simulink model "Cerano23210696Pr4"  (R2023a)
settings: Solver=ode15s  StartTime=0.0  StopTime=10.0  MaxStep=1E-3  RelTol=1e-3
libraries: fl_lib x14, nesl_utility x6, slpidlib x1
settings Model: LastModifiedBy=David
settings DataIOCC: SaveFormat=Array  ReturnWorkspaceOutputs=off  TimeSaveName=t
settings DebuggingCC: AlgebraicLoopMsg=none  ArtificialAlgebraicLoopMsg=none  MaxConsecutiveZCsMsg=none  ModelReferenceExtraNoncontSigs=none  OperatingPointInterfaceChecksumMismatchMsg=none
settings RTWCC: GPUComputeCapability=5.0

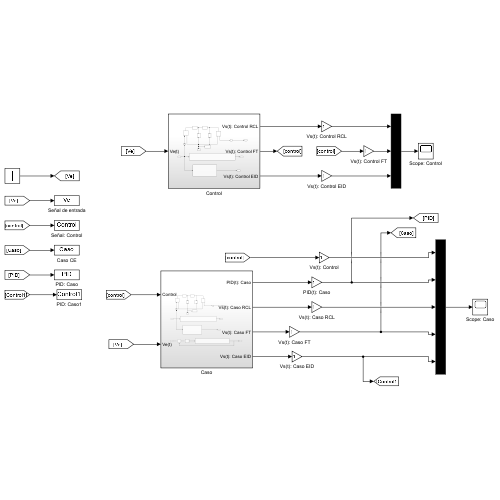
[thumbnail: Simulink's stored preview of the top-level diagram]
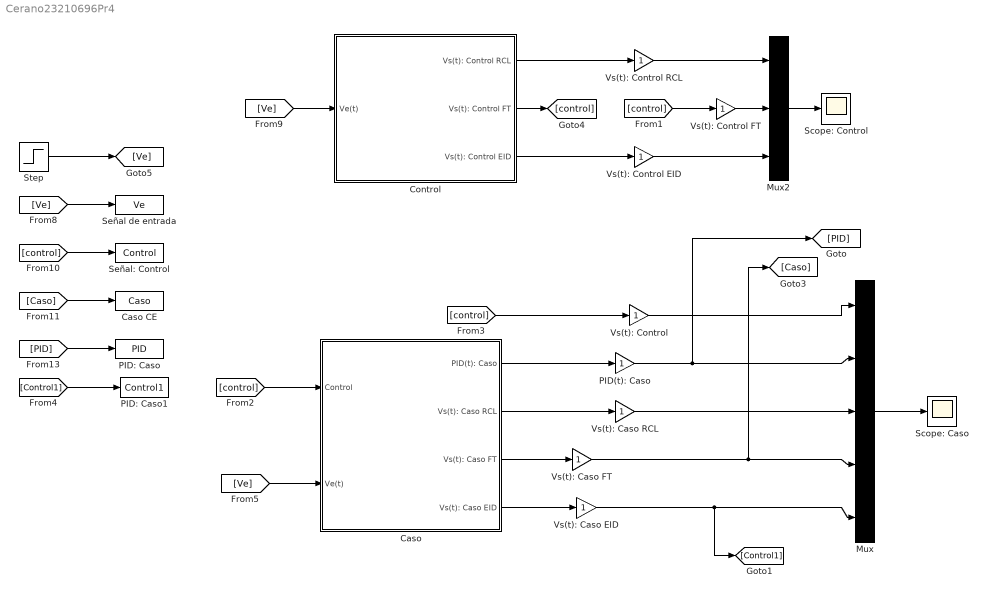
== system Cerano23210696Pr4 ==
  Caso : Subsystem
  Caso CE : ToWorkspace  VariableName=Caso  SampleTime=-1
  Control : Subsystem
  Mux : Mux  Inputs=5
  Mux2 : Mux  Inputs=3
  PID(t): Caso : Gain
  PID: Caso : ToWorkspace  VariableName=PID  SampleTime=-1
  PID: Caso1 : ToWorkspace  VariableName=Control1  SampleTime=-1
  Scope: Caso : Scope
  Scope: Control : Scope
  Señal de entrada : ToWorkspace  VariableName=Ve  SampleTime=-1
  Señal: Control : ToWorkspace  VariableName=Control  SampleTime=-1
  Step : Step  Time=0  SampleTime=0
  Vs(t): Caso EID : Gain
  Vs(t): Caso FT : Gain
  Vs(t): Caso RCL : Gain
  Vs(t): Control : Gain
  Vs(t): Control EID : Gain
  Vs(t): Control FT : Gain
  Vs(t): Control RCL : Gain
  wires:
  Mux/1 -> Scope: Caso/1
  [control] -> Caso/1(Control)
  [Ve] -> Caso/2(Ve(t))
  Mux2/1 -> Scope: Control/1
  [control] -> Vs(t): Control FT/1
  [Ve] -> Señal de entrada/1
  [control] -> Señal: Control/1
  [Caso] -> Caso CE/1
  [PID] -> PID: Caso/1
  Step/1 -> [Ve]
  Vs(t): Control FT/1 -> Mux2/2
  Vs(t): Control RCL/1 -> Mux2/1
  Control/1(Vs(t): Control RCL) -> Vs(t): Control RCL/1
  Control/2(Vs(t): Control FT) -> [control]
  [Ve] -> Control/1(Ve(t))
  Control/3(Vs(t): Control EID) -> Vs(t): Control EID/1
  Vs(t): Control EID/1 -> Mux2/3
  [control] -> Vs(t): Control/1
  Vs(t): Control/1 -> Mux/1
  Caso/2(Vs(t): Caso RCL) -> Vs(t): Caso RCL/1
  Vs(t): Caso RCL/1 -> Mux/3
  Caso/1(PID(t): Caso) -> PID(t): Caso/1
  PID(t): Caso/1 -> [PID], Mux/2
  Caso/3(Vs(t): Caso FT) -> Vs(t): Caso FT/1
  Caso/4(Vs(t): Caso EID) -> Vs(t): Caso EID/1
  Vs(t): Caso EID/1 -> [Control1], Mux/5
  Vs(t): Caso FT/1 -> [Caso], Mux/4
  [Control1] -> PID: Caso1/1

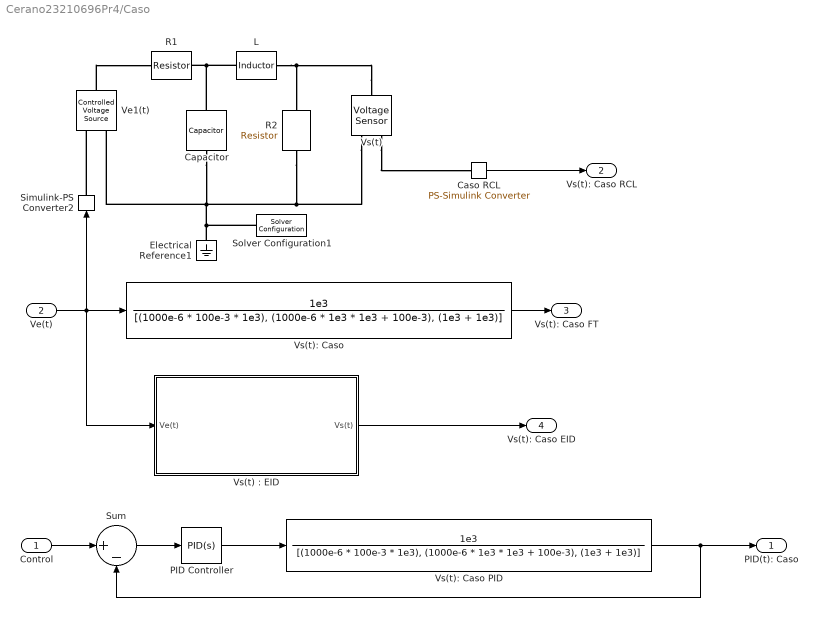
== system Cerano23210696Pr4/Caso ==
  Control : Inport
  Ve(t) : Inport  Port=2
  Capacitor : fl_lib/Electrical/Electrical Elements/Capacitor  c=1000 uF  r=1e-6 Ohm  g=0 1/Ohm  i_specify=off  i_priority=None  i=0 A  i_nominal_specify=off  i_nominal_unit=A  i_nominal_value=1  v_specify=off  v_priority=None  v=0 V  v_nominal_specify=off  v_nominal_unit=V  v_nominal_value=1  vc_specify=off  vc_priority=High  vc=0 V  vc_nominal_specify=off  vc_nominal_unit=V  vc_nominal_value=1
  Caso RCL : nesl_utility/PS-Simulink Converter  PhysicalDomain=network_engine_domain  SubClassName=ps_output  LeftPortType=input  RightPortType=output  PseudoPeriodic=off  Frequencies=[]  VectorFormat=1-D array  Unit=inherit  AffineConversion=off
  Electrical Reference1 : fl_lib/Electrical/Electrical Elements/Electrical Reference
  L : fl_lib/Electrical/Electrical Elements/Inductor  l=100 mH  r=0 Ohm  g=1e-9 1/Ohm  i_specify=off  i_priority=None  i=0 A  i_nominal_specify=off  i_nominal_unit=A  i_nominal_value=1  v_specify=off  v_priority=None  v=0 V  v_nominal_specify=off  v_nominal_unit=V  v_nominal_value=1  i_L_specify=off  i_L_priority=High  i_L=0 A  i_L_nominal_specify=off  i_L_nominal_unit=A  i_L_nominal_value=1
  PID Controller : slpidlib/PID Controller  Controller=PID  Form=Parallel  TimeDomain=Continuous-time  UseExternalTs=off  SampleTime=-1  IntegratorMethod=Forward Euler  FilterMethod=Forward Euler  ControllerParametersSource=internal  P=139.024398952871  I=3579.00250163921  UseKiTs=off  D=0.182003845761544  N=531.620758823067  UseFilter=on  TunerSelectOption=Transfer Function Based (PID Tuner App)  InitialConditionSource=internal  InitialConditionForIntegrator=0  InitialConditionForFilter=0  DifferentiatorICPrevScaledInput=0  ExternalReset=none  TrackingMode=off  Kt=1  LimitOutput=off  SatLimitsSource=internal  UpperSaturationLimit=inf  LowerSaturationLimit=-inf  LinearizeAsGain=on  AntiWindupMode=none  Kb=1  LimitIntegrator=off  UpperIntegratorSaturationLimit=inf  LowerIntegratorSaturationLimit=-inf  POutMin=[]  POutMax=[]  IOutMin=[]  IOutMax=[]  DOutMin=[]  DOutMax=[]  NOutMin=[]  NOutMax=[]  SumOutMin=[]  SumOutMax=[]  SaturationOutMin=[]  SaturationOutMax=[]  PParamMin=[]  PParamMax=[]  IParamMin=[]  IParamMax=[]  DParamMin=[]  DParamMax=[]  NParamMin=[]  NParamMax=[]  KbParamMin=[]  KbParamMax=[]  KtParamMin=[]  KtParamMax=[]  KbOutMin=[]  KbOutMax=[]  KtOutMin=[]  KtOutMax=[]  IntegratorOutMin=[]  IntegratorOutMax=[]  FilterOutMin=[]  FilterOutMax=[]  SumI1OutMin=[]  SumI1OutMax=[]  SumI2OutMin=[]  SumI2OutMax=[]  SumI3OutMin=[]  SumI3OutMax=[]  SumI4OutMin=[]  SumI4OutMax=[]  SumDOutMin=[]  SumDOutMax=[]  DifferentiatorOutMin=[]  DifferentiatorOutMax=[]  FilterDiffOutCoefMin=[]  FilterDiffOutCoefMax=[]  ReciprocalOutMin=[]  ReciprocalOutMax=[]  SumDenOutMin=[]  SumDenOutMax=[]  SumNumOutMin=[]  SumNumOutMax=[]  DivideOutMin=[]  DivideOutMax=[]  UdiffTsProdOutMin=[]  UdiffTsProdOutMax=[]  NTsProdOutMin=[]  NTsProdOutMax=[]  UintegralTsProdOutMin=[]  UintegralTsProdOutMax=[]  UngainTsProdOutMin=[]  UngainTsProdOutMax=[]  ClampingZeroOutDataTypeStr=Inherit: Inherit via back propagation  ClampingZeroOutMin=[]  ClampingZeroOutMax=[]  FilterDenConstantOutDataTypeStr=Inherit: Inherit via back propagation  FilterDenConstantOutMin=[]  FilterDenConstantOutMax=[]  PCopyOutDataTypeStr=Inherit: Inherit via back propagation  PCopyOutMin=[]  PCopyOutMax=[]  NCopyOutDataTypeStr=Inherit: Inherit via back propagation  NCopyOutMin=[]  NCopyOutMax=[]  IntegratorContinuousStateAttributes=''  IntegratorStateMustResolveToSignalObject=off  IntegratorRTWStateStorageClass=Auto  FilterContinuousStateAttributes=''  FilterStateMustResolveToSignalObject=off  FilterRTWStateStorageClass=Auto  ParallelPVariant=InternalParameters  IdealPVariant=Disabled  IVariant=InternalParameters  DVariant=InternalParameters  IntegratorVariant=Continuous  SatVariant=Disabled  AWVariant=Passthrough  PCopyVariant=Disabled  TRVariant=Disabled  FdbkBlocksVariant=Forward  IdealPFdbkVariant=Disabled  SatFdbkVariant=Disabled  DerivativeFilterVariant=ContFilter  NVariant=InternalParameters  NCopyVariant=Disabled  FilterICVariant=InternalICsFilter  IntegratorICVariant=InternalICs  ExternalResetVariant=Disabled  TRSumVariant=Passthrough  SumFdbkVariant=Disabled  SumVariant=Sum_PID  TsampFilterVariant=InternalTs  TsampNgainVariant=Passthrough  TsampIntegralVariant=Disabled_SignalSpec  ExternalSaturationOutDataTypeStr=Inherit: Same as second input
  R1 : fl_lib/Electrical/Electrical Elements/Resistor  R=1 kOhm  i_specify=off  i_priority=None  i=0 A  i_nominal_specify=off  i_nominal_unit=A  i_nominal_value=1  v_specify=off  v_priority=None  v=0 V  v_nominal_specify=off  v_nominal_unit=V  v_nominal_value=1
  R2 : fl_lib/Electrical/Electrical Elements/Resistor  R=1 kOhm  i_specify=off  i_priority=None  i=0 A  i_nominal_specify=off  i_nominal_unit=A  i_nominal_value=1  v_specify=off  v_priority=None  v=0 V  v_nominal_specify=off  v_nominal_unit=V  v_nominal_value=1
  Simulink-PS Converter2 : nesl_utility/Simulink-PS Converter  PhysicalDomain=network_engine_domain  SubClassName=ps_input  LeftPortType=input  RightPortType=output  PseudoPeriodic=off  Frequencies=[]  NoiseDistribution=none  NoiseParameters=[]  Unit=1  AffineConversion=off  FilteringAndDerivatives=provide  SimscapeFilterOrder=1  InputFilterTimeConstant=0.001  UdotUserProvided=0
  Solver Configuration1 : nesl_utility/Solver Configuration  PhysicalDomain=network_engine_domain  SubClassName=solver  LeftPortType=input  RightPortType=generic  Tones=[]  Harmonics=[]  SimulateNoise=off  Profile=off  UseLocalSampling=off  EnableSwitchedLinearOptims=on  FrequencyDomain=off  UseCCode=off  RelTol=0.001  AbsTol=0.001  MinStep=1e-09  ToWorkspace=off  RevertToSquareIcSolve=off  NumHomotopyIterations=100  PhasorMode=off  PhasorModeNumHarmonics=1  ConsistencySolver=NEWTON_XTOL_AFTER_FTOL  IndexReductionMethod=DerivativeReplacement  DoDC=off  ResidualTolerance=1e-09  ConsistencyTolSource=GLOBAL  ConsistencyAbsTol=0.001  ConsistencyRelTol=0.001  ConsistencyTolFactor=0.001  UseLocalSolver=off  LocalSolverChoice=NE_BACKWARD_EULER_ADVANCER  ResolveIndetEquations=on  FunctionEvalNumThread=1  LocalSolverSampleTime=0.001  DoFixedCost=off  MaxNonlinIter=3  MaxModeIter=2  ComputeImpulses=off  ImpulseIterations=2  LinearAlgebra=auto  LinearAlgebraNumThread=0  EquationFormulation=NE_TIME_EF  DelaysMemoryBudget=1024  AutomaticFiltering=on  FilteringTimeConstant=0.001  PartitionStorageMethod=AS_NEEDED  PartitionMemoryBudget=1024  PartitionMethod=ROBUST
  Sum : Sum  Inputs=|+-
  Ve1(t) : fl_lib/Electrical/Electrical Sources/Controlled Voltage Source
  Vs(t) : fl_lib/Electrical/Electrical Sensors/Voltage Sensor
  "Vs(t) : EID" : Subsystem
  Vs(t): Caso : TransferFcn  Numerator=[1e3]  Denominator=[(1000e-6 * 100e-3 * 1e3), (1000e-6 * 1e3 * 1e3 + 100e-3), (1e3 + 1e3)]
  Vs(t): Caso PID : TransferFcn  Numerator=[1e3]  Denominator=[(1000e-6 * 100e-3 * 1e3), (1000e-6 * 1e3 * 1e3 + 100e-3), (1e3 + 1e3)]
  PID(t): Caso : Outport
  Vs(t): Caso RCL : Outport  Port=2
  Vs(t): Caso FT : Outport  Port=3
  Vs(t): Caso EID : Outport  Port=4
  wires:
  Sum/1 -> PID Controller/1
  Vs(t): Caso PID/1 -> PID(t): Caso/1, Sum/2
  PID Controller/1 -> Vs(t): Caso PID/1
  Control/1 -> Sum/1
  Vs(t): Caso/1 -> Vs(t): Caso FT/1
  "Vs(t) : EID"/1(Vs(t)) -> Vs(t): Caso EID/1
  Ve(t)/1 -> "Vs(t) : EID"/1(Ve(t)), Simulink-PS Converter2/1, Vs(t): Caso/1
  Caso RCL/1 -> Vs(t): Caso RCL/1
  connections:
  R2/LConn1 -- Vs(t)/RConn2 -- Capacitor/RConn1 -- Electrical Reference1/LConn1 -- Solver Configuration1/RConn1 -- Ve1(t)/RConn2
  Vs(t)/LConn1 -- L/RConn1 -- R2/RConn1
  R1/LConn1 -- Capacitor/LConn1 -- L/LConn1
  Ve1(t)/LConn1 -- R1/RConn1
  Vs(t)/RConn1 -- Caso RCL/LConn1
  Simulink-PS Converter2/RConn1 -- Ve1(t)/RConn1

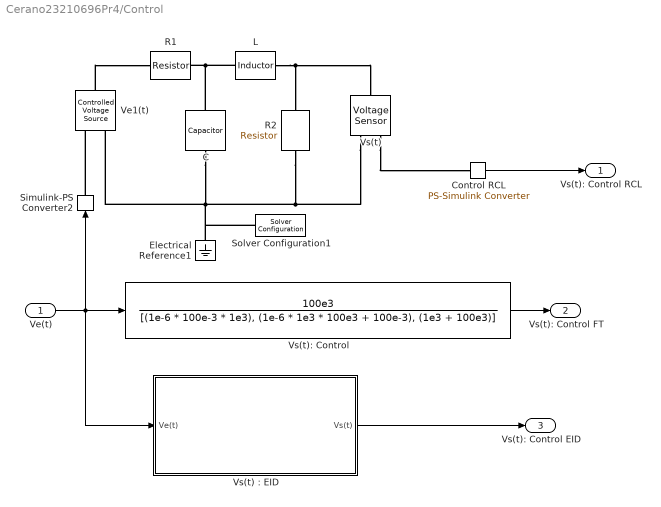
== system Cerano23210696Pr4/Control ==
  Ve(t) : Inport
  C : fl_lib/Electrical/Electrical Elements/Capacitor  c=1 uF  r=1e-6 Ohm  g=0 1/Ohm  i_specify=off  i_priority=None  i=0 A  i_nominal_specify=off  i_nominal_unit=A  i_nominal_value=1  v_specify=off  v_priority=None  v=0 V  v_nominal_specify=off  v_nominal_unit=V  v_nominal_value=1  vc_specify=off  vc_priority=High  vc=0 V  vc_nominal_specify=off  vc_nominal_unit=V  vc_nominal_value=1
  Control RCL : nesl_utility/PS-Simulink Converter  PhysicalDomain=network_engine_domain  SubClassName=ps_output  LeftPortType=input  RightPortType=output  PseudoPeriodic=off  Frequencies=[]  VectorFormat=1-D array  Unit=inherit  AffineConversion=off
  Electrical Reference1 : fl_lib/Electrical/Electrical Elements/Electrical Reference
  L : fl_lib/Electrical/Electrical Elements/Inductor  l=100 mH  r=0 Ohm  g=1e-9 1/Ohm  i_specify=off  i_priority=None  i=0 A  i_nominal_specify=off  i_nominal_unit=A  i_nominal_value=1  v_specify=off  v_priority=None  v=0 V  v_nominal_specify=off  v_nominal_unit=V  v_nominal_value=1  i_L_specify=off  i_L_priority=High  i_L=0 A  i_L_nominal_specify=off  i_L_nominal_unit=A  i_L_nominal_value=1
  R1 : fl_lib/Electrical/Electrical Elements/Resistor  R=1 kOhm  i_specify=off  i_priority=None  i=0 A  i_nominal_specify=off  i_nominal_unit=A  i_nominal_value=1  v_specify=off  v_priority=None  v=0 V  v_nominal_specify=off  v_nominal_unit=V  v_nominal_value=1
  R2 : fl_lib/Electrical/Electrical Elements/Resistor  R=100 kOhm  i_specify=off  i_priority=None  i=0 A  i_nominal_specify=off  i_nominal_unit=A  i_nominal_value=1  v_specify=off  v_priority=None  v=0 V  v_nominal_specify=off  v_nominal_unit=V  v_nominal_value=1
  Simulink-PS Converter2 : nesl_utility/Simulink-PS Converter  PhysicalDomain=network_engine_domain  SubClassName=ps_input  LeftPortType=input  RightPortType=output  PseudoPeriodic=off  Frequencies=[]  NoiseDistribution=none  NoiseParameters=[]  Unit=1  AffineConversion=off  FilteringAndDerivatives=provide  SimscapeFilterOrder=1  InputFilterTimeConstant=0.001  UdotUserProvided=0
  Solver Configuration1 : nesl_utility/Solver Configuration  PhysicalDomain=network_engine_domain  SubClassName=solver  LeftPortType=input  RightPortType=generic  Tones=[]  Harmonics=[]  SimulateNoise=off  Profile=off  UseLocalSampling=off  EnableSwitchedLinearOptims=on  FrequencyDomain=off  UseCCode=off  RelTol=0.001  AbsTol=0.001  MinStep=1e-09  ToWorkspace=off  RevertToSquareIcSolve=off  NumHomotopyIterations=100  PhasorMode=off  PhasorModeNumHarmonics=1  ConsistencySolver=NEWTON_XTOL_AFTER_FTOL  IndexReductionMethod=DerivativeReplacement  DoDC=off  ResidualTolerance=1e-09  ConsistencyTolSource=GLOBAL  ConsistencyAbsTol=0.001  ConsistencyRelTol=0.001  ConsistencyTolFactor=0.001  UseLocalSolver=off  LocalSolverChoice=NE_BACKWARD_EULER_ADVANCER  ResolveIndetEquations=on  FunctionEvalNumThread=1  LocalSolverSampleTime=0.001  DoFixedCost=off  MaxNonlinIter=3  MaxModeIter=2  ComputeImpulses=off  ImpulseIterations=2  LinearAlgebra=auto  LinearAlgebraNumThread=0  EquationFormulation=NE_TIME_EF  DelaysMemoryBudget=1024  AutomaticFiltering=on  FilteringTimeConstant=0.001  PartitionStorageMethod=AS_NEEDED  PartitionMemoryBudget=1024  PartitionMethod=ROBUST
  Ve1(t) : fl_lib/Electrical/Electrical Sources/Controlled Voltage Source
  Vs(t) : fl_lib/Electrical/Electrical Sensors/Voltage Sensor
  "Vs(t) : EID" : Subsystem
  Vs(t): Control : TransferFcn  Numerator=[100e3]  Denominator=[(1e-6 * 100e-3 * 1e3), (1e-6 * 1e3 * 100e3 + 100e-3), (1e3 + 100e3)]
  Vs(t): Control RCL : Outport
  Vs(t): Control FT : Outport  Port=2
  Vs(t): Control EID : Outport  Port=3
  wires:
  Control RCL/1 -> Vs(t): Control RCL/1
  Ve(t)/1 -> "Vs(t) : EID"/1(Ve(t)), Simulink-PS Converter2/1, Vs(t): Control/1
  Vs(t): Control/1 -> Vs(t): Control FT/1
  "Vs(t) : EID"/1(Vs(t)) -> Vs(t): Control EID/1
  connections:
  Ve1(t)/LConn1 -- R1/RConn1
  L/RConn1 -- R2/RConn1 -- Vs(t)/LConn1
  Vs(t)/RConn2 -- Electrical Reference1/LConn1 -- Solver Configuration1/RConn1 -- Ve1(t)/RConn2 -- C/RConn1 -- R2/LConn1
  Vs(t)/RConn1 -- Control RCL/LConn1
  Simulink-PS Converter2/RConn1 -- Ve1(t)/RConn1
  C/LConn1 -- L/LConn1 -- R1/LConn1

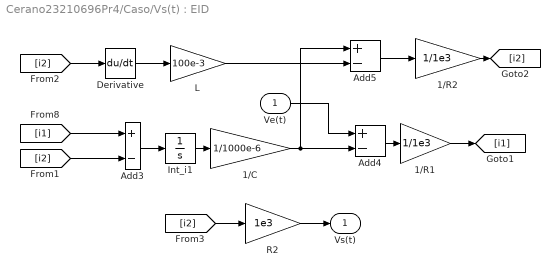
== system Cerano23210696Pr4/Caso/Vs(t) : EID ==
  Ve(t) : Inport
  1/C : Gain  Gain=1/1000e-6
  1/R1 : Gain  Gain=1/1e3
  1/R2 : Gain  Gain=1/1e3
  Add3 : Sum  Inputs=+-
  Add4 : Sum  Inputs=+-
  Add5 : Sum  Inputs=+-
  Derivative : Derivative
  Int_i1 : Integrator
  L : Gain  Gain=100e-3
  R2 : Gain  Gain=1e3
  Vs(t) : Outport
  wires:
  [i1] -> Add3/1
  [i2] -> Add3/2
  Add3/1 -> Int_i1/1
  Int_i1/1 -> 1/C/1
  1/C/1 -> Add5/1, Add4/2
  Ve(t)/1 -> Add4/1
  Add4/1 -> 1/R1/1
  1/R1/1 -> [i1]
  [i2] -> Derivative/1
  Derivative/1 -> L/1
  L/1 -> Add5/2
  Add5/1 -> 1/R2/1
  1/R2/1 -> [i2]
  [i2] -> R2/1
  R2/1 -> Vs(t)/1

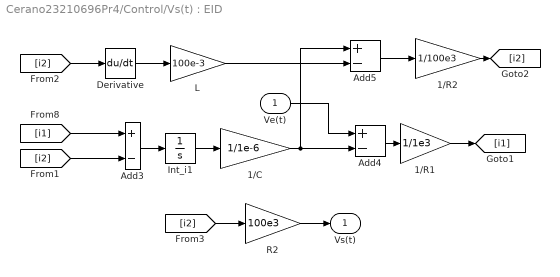
== system Cerano23210696Pr4/Control/Vs(t) : EID ==
  Ve(t) : Inport
  1/C : Gain  Gain=1/1e-6
  1/R1 : Gain  Gain=1/1e3
  1/R2 : Gain  Gain=1/100e3
  Add3 : Sum  Inputs=+-
  Add4 : Sum  Inputs=+-
  Add5 : Sum  Inputs=+-
  Derivative : Derivative
  Int_i1 : Integrator
  L : Gain  Gain=100e-3
  R2 : Gain  Gain=100e3
  Vs(t) : Outport
  wires:
  [i1] -> Add3/1
  [i2] -> Add3/2
  Add3/1 -> Int_i1/1
  Int_i1/1 -> 1/C/1
  1/C/1 -> Add5/1, Add4/2
  Ve(t)/1 -> Add4/1
  Add4/1 -> 1/R1/1
  1/R1/1 -> [i1]
  [i2] -> Derivative/1
  Derivative/1 -> L/1
  L/1 -> Add5/2
  Add5/1 -> 1/R2/1
  1/R2/1 -> [i2]
  [i2] -> R2/1
  R2/1 -> Vs(t)/1
